simulink model "PruebasKUF_Envolvente"  (R2026a)
settings: Solver=VariableStepAuto  StopTime=10  MaxStep=0.01
values from neighbouring files (symbols this model uses):
  B = -c.b*I/r^2    [ComparacionKUF.m]
  g = 9.81    [ComparacionKUF.m]    (also in DespejeKuf.m)
  I = 3.2*382.232e-7    (= 0.00012231424)    [ComparacionKUF.m]
  lc = 40.67e-3    (= 0.04067)    [ComparacionKUF.m]    (also in DespejeKuf.m = 0.040677)
  m = 30.00e-3    (= 0.03)    [ComparacionKUF.m]    (also in DespejeKuf.m)
  r = 135.0e-3    (= 0.135)    [ComparacionKUF.m]    (also in DespejeKuf.m)
settings Model: Creator=sslan  LastModifiedBy=leonardoa29

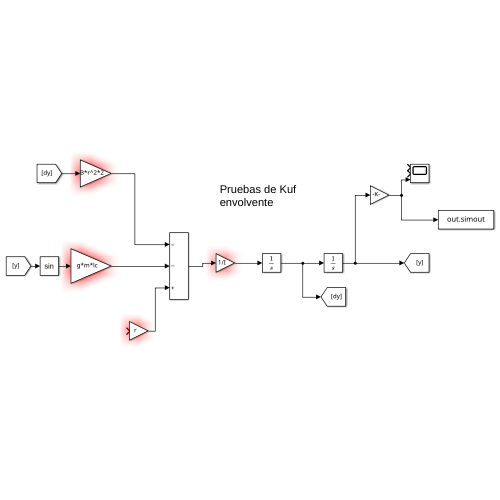
[thumbnail: Simulink's stored preview of the top-level diagram]
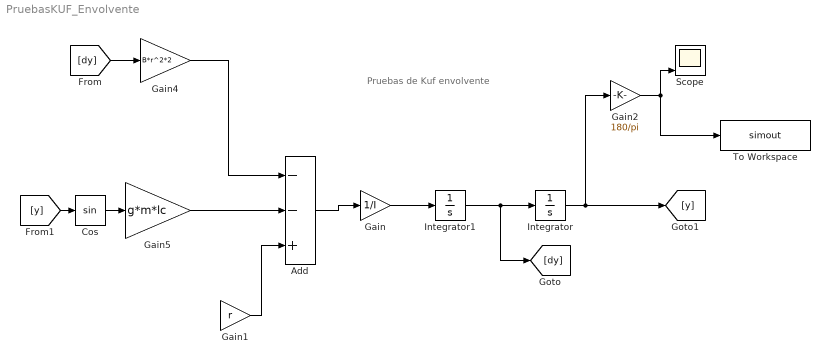
== system PruebasKUF_Envolvente ==
  note: Pruebas de Kuf envolvente
  Add : Sum  Inputs=--+
  Cos : Trigonometry
  Gain : Gain  Gain=1/I
  Gain1 : Gain  Gain=r
  Gain2 : Gain  Gain=180/pi
  Gain4 : Gain  Gain=B*r^2*2
  Gain5 : Gain  Gain=g*m*lc
  Integrator : Integrator  InitialCondition=pi/2
  Integrator1 : Integrator
  Scope : Scope  NumInputPorts=3
      settings: ActiveDisplayYMinimum=-0.80347256770612918  ActiveDisplayYMaximum=0.68895822556712538
  To Workspace : ToWorkspace  VariableName=simout  SaveFormat=Timeseries  SampleTime=-1
  wires:
  Gain5/1 -> Add/2
  Cos/1 -> Gain5/1
  Integrator/1 -> [y], Gain2/1
  Gain/1 -> Integrator1/1
  [y] -> Cos/1
  Integrator1/1 -> [dy], Integrator/1
  [dy] -> Gain4/1
  Gain2/1 -> Scope/3, To Workspace/1
  Gain1/1 -> Add/3
  Gain4/1 -> Add/1
  Add/1 -> Gain/1
